simulink model "draw_aircraft_sim"  (R2024a)
settings: Solver=FixedStepDiscrete  StartTime=0.0  StopTime=1E4  FixedStep=0.1  RelTol=1e-3
libraries: simulink x8
settings Model: Creator=pf  LastModifiedBy=pf
settings RTWCC: GPUComputeCapability=3.5

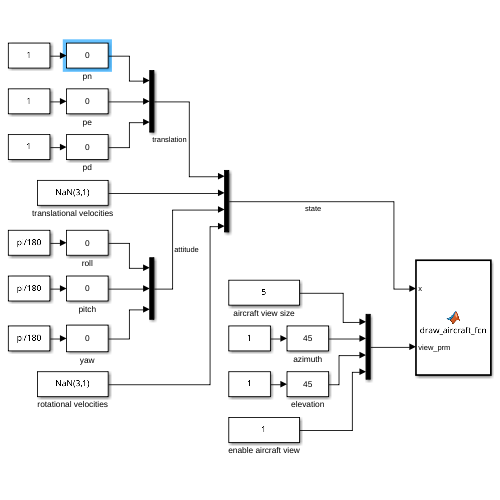
[thumbnail: Simulink's stored preview of the top-level diagram]
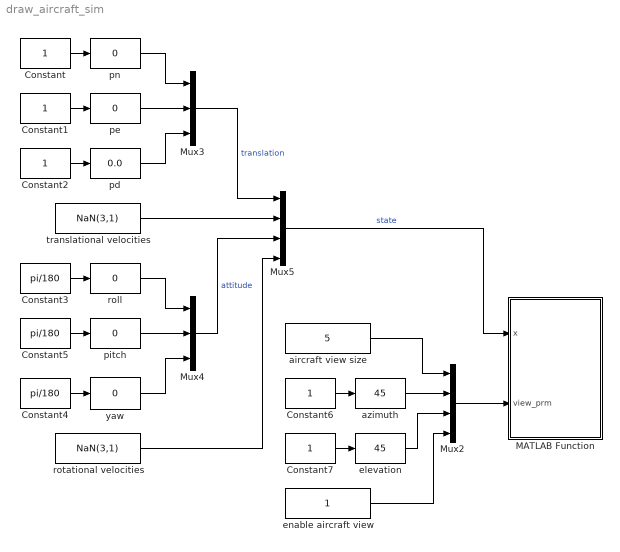
== system draw_aircraft_sim ==
  Constant{,1..2,6..7} (5 alike) : Constant
  Constant3 : Constant  Value=pi/180
  Constant4 : Constant  Value=pi/180
  Constant5 : Constant  Value=pi/180
  MATLAB Function : MATLAB Function  TreatAsAtomicUnit=on
  Mux2 : Mux
  Mux3 : Mux  Inputs=3
  Mux4 : Mux  Inputs=3
  Mux5 : Mux
  aircraft view size : Constant  Value=5
  azimuth : simulink/Math Operations/Slider Gain  gain=45  low=-180  high=180
  elevation : simulink/Math Operations/Slider Gain  gain=45  low=-180  high=180
  enable aircraft view : Constant
  pd : simulink/Math Operations/Slider Gain  gain=0.0  low=-12  high=12
  pe : simulink/Math Operations/Slider Gain  gain=0  low=-12  high=12
  pitch : simulink/Math Operations/Slider Gain  gain=0  low=-90  high=90
  pn : simulink/Math Operations/Slider Gain  gain=0  low=-12  high=12
  roll : simulink/Math Operations/Slider Gain  gain=0  low=-180  high=180
  rotational velocities : Constant  Value=NaN(3,1)
  translational velocities : Constant  Value=NaN(3,1)
  yaw : simulink/Math Operations/Slider Gain  gain=0  low=-180  high=180
  wires:
  Constant/1 -> pn/1
  Constant1/1 -> pe/1
  Constant2/1 -> pd/1
  pn/1 -> Mux3/1
  pe/1 -> Mux3/2
  pd/1 -> Mux3/3
  Constant3/1 -> roll/1
  roll/1 -> Mux4/1
  Constant4/1 -> yaw/1
  Constant5/1 -> pitch/1
  pitch/1 -> Mux4/2
  yaw/1 -> Mux4/3
  translational velocities/1 -> Mux5/2
  Mux3/1 -> Mux5/1  "translation"
  Mux4/1 -> Mux5/3  "attitude"
  rotational velocities/1 -> Mux5/4
  Mux5/1 -> MATLAB Function/1(x)  "state"
  Constant6/1 -> azimuth/1
  Constant7/1 -> elevation/1
  aircraft view size/1 -> Mux2/1
  Mux2/1 -> MATLAB Function/2(view_prm)
  azimuth/1 -> Mux2/2
  elevation/1 -> Mux2/3
  enable aircraft view/1 -> Mux2/4

== matlab function draw_aircraft_sim/MATLAB Function ==
  data: x input; view_prm input
function draw_aircraft_fcn(x,view_prm)
    draw_aircraft(x,view_prm);
end
